simulink model "s_c_nbe_m32k"  (R2018a)
settings: Solver=VariableStepDiscrete  StartTime=0.0  StopTime=1000  RelTol=1e-3
undefined symbols (not defined in the file): fft_stages, n_taps, output_bits, pfb_coeff_gen_calc, xengbits
libraries: xbsIndex_r4 x23714, casper_library_misc x17, xps_library x4, casper_library_scopes x4, xbsReplacements_r4 x4
(part 152 of 171)

== system s_c_nbe_m32k/nb_pfb/pfb_fir_generic1/pfb_fir_taps/tap_delays/debus_web0 ==
  bus_in : Inport
  slice1 : xbsIndex_r4/Slice  nbits=1  boolean_output=on  mode=Upper Bit Location + Width  bit1=-107  base1=MSB of Input  bit0=0  base0=LSB of Input  dbl_ovrd=off  block_type=slice
  slice10 : xbsIndex_r4/Slice  nbits=1  boolean_output=on  mode=Upper Bit Location + Width  bit1=-98  base1=MSB of Input  bit0=0  base0=LSB of Input  dbl_ovrd=off  block_type=slice
  slice100 : xbsIndex_r4/Slice  nbits=1  boolean_output=on  mode=Upper Bit Location + Width  bit1=-8  base1=MSB of Input  bit0=0  base0=LSB of Input  dbl_ovrd=off  block_type=slice
  slice101 : xbsIndex_r4/Slice  nbits=1  boolean_output=on  mode=Upper Bit Location + Width  bit1=-7  base1=MSB of Input  bit0=0  base0=LSB of Input  dbl_ovrd=off  block_type=slice
  slice102 : xbsIndex_r4/Slice  nbits=1  boolean_output=on  mode=Upper Bit Location + Width  bit1=-6  base1=MSB of Input  bit0=0  base0=LSB of Input  dbl_ovrd=off  block_type=slice
  slice103 : xbsIndex_r4/Slice  nbits=1  boolean_output=on  mode=Upper Bit Location + Width  bit1=-5  base1=MSB of Input  bit0=0  base0=LSB of Input  dbl_ovrd=off  block_type=slice
  slice104 : xbsIndex_r4/Slice  nbits=1  boolean_output=on  mode=Upper Bit Location + Width  bit1=-4  base1=MSB of Input  bit0=0  base0=LSB of Input  dbl_ovrd=off  block_type=slice
  slice105 : xbsIndex_r4/Slice  nbits=1  boolean_output=on  mode=Upper Bit Location + Width  bit1=-3  base1=MSB of Input  bit0=0  base0=LSB of Input  dbl_ovrd=off  block_type=slice
  slice106 : xbsIndex_r4/Slice  nbits=1  boolean_output=on  mode=Upper Bit Location + Width  bit1=-2  base1=MSB of Input  bit0=0  base0=LSB of Input  dbl_ovrd=off  block_type=slice
  slice107 : xbsIndex_r4/Slice  nbits=1  boolean_output=on  mode=Upper Bit Location + Width  bit1=-1  base1=MSB of Input  bit0=0  base0=LSB of Input  dbl_ovrd=off  block_type=slice
  slice108 : xbsIndex_r4/Slice  nbits=1  boolean_output=on  mode=Upper Bit Location + Width  bit1=0  base1=MSB of Input  bit0=0  base0=LSB of Input  dbl_ovrd=off  block_type=slice
  slice11 : xbsIndex_r4/Slice  nbits=1  boolean_output=on  mode=Upper Bit Location + Width  bit1=-97  base1=MSB of Input  bit0=0  base0=LSB of Input  dbl_ovrd=off  block_type=slice
  slice12 : xbsIndex_r4/Slice  nbits=1  boolean_output=on  mode=Upper Bit Location + Width  bit1=-96  base1=MSB of Input  bit0=0  base0=LSB of Input  dbl_ovrd=off  block_type=slice
  slice13 : xbsIndex_r4/Slice  nbits=1  boolean_output=on  mode=Upper Bit Location + Width  bit1=-95  base1=MSB of Input  bit0=0  base0=LSB of Input  dbl_ovrd=off  block_type=slice
  slice14 : xbsIndex_r4/Slice  nbits=1  boolean_output=on  mode=Upper Bit Location + Width  bit1=-94  base1=MSB of Input  bit0=0  base0=LSB of Input  dbl_ovrd=off  block_type=slice
  slice15 : xbsIndex_r4/Slice  nbits=1  boolean_output=on  mode=Upper Bit Location + Width  bit1=-93  base1=MSB of Input  bit0=0  base0=LSB of Input  dbl_ovrd=off  block_type=slice
  slice16 : xbsIndex_r4/Slice  nbits=1  boolean_output=on  mode=Upper Bit Location + Width  bit1=-92  base1=MSB of Input  bit0=0  base0=LSB of Input  dbl_ovrd=off  block_type=slice
  slice17 : xbsIndex_r4/Slice  nbits=1  boolean_output=on  mode=Upper Bit Location + Width  bit1=-91  base1=MSB of Input  bit0=0  base0=LSB of Input  dbl_ovrd=off  block_type=slice
  slice18 : xbsIndex_r4/Slice  nbits=1  boolean_output=on  mode=Upper Bit Location + Width  bit1=-90  base1=MSB of Input  bit0=0  base0=LSB of Input  dbl_ovrd=off  block_type=slice
  slice19 : xbsIndex_r4/Slice  nbits=1  boolean_output=on  mode=Upper Bit Location + Width  bit1=-89  base1=MSB of Input  bit0=0  base0=LSB of Input  dbl_ovrd=off  block_type=slice
  slice2 : xbsIndex_r4/Slice  nbits=1  boolean_output=on  mode=Upper Bit Location + Width  bit1=-106  base1=MSB of Input  bit0=0  base0=LSB of Input  dbl_ovrd=off  block_type=slice
  slice20 : xbsIndex_r4/Slice  nbits=1  boolean_output=on  mode=Upper Bit Location + Width  bit1=-88  base1=MSB of Input  bit0=0  base0=LSB of Input  dbl_ovrd=off  block_type=slice
  slice21 : xbsIndex_r4/Slice  nbits=1  boolean_output=on  mode=Upper Bit Location + Width  bit1=-87  base1=MSB of Input  bit0=0  base0=LSB of Input  dbl_ovrd=off  block_type=slice
  slice22 : xbsIndex_r4/Slice  nbits=1  boolean_output=on  mode=Upper Bit Location + Width  bit1=-86  base1=MSB of Input  bit0=0  base0=LSB of Input  dbl_ovrd=off  block_type=slice
  slice23 : xbsIndex_r4/Slice  nbits=1  boolean_output=on  mode=Upper Bit Location + Width  bit1=-85  base1=MSB of Input  bit0=0  base0=LSB of Input  dbl_ovrd=off  block_type=slice
  slice24 : xbsIndex_r4/Slice  nbits=1  boolean_output=on  mode=Upper Bit Location + Width  bit1=-84  base1=MSB of Input  bit0=0  base0=LSB of Input  dbl_ovrd=off  block_type=slice
  slice25 : xbsIndex_r4/Slice  nbits=1  boolean_output=on  mode=Upper Bit Location + Width  bit1=-83  base1=MSB of Input  bit0=0  base0=LSB of Input  dbl_ovrd=off  block_type=slice
  slice26 : xbsIndex_r4/Slice  nbits=1  boolean_output=on  mode=Upper Bit Location + Width  bit1=-82  base1=MSB of Input  bit0=0  base0=LSB of Input  dbl_ovrd=off  block_type=slice
  slice27 : xbsIndex_r4/Slice  nbits=1  boolean_output=on  mode=Upper Bit Location + Width  bit1=-81  base1=MSB of Input  bit0=0  base0=LSB of Input  dbl_ovrd=off  block_type=slice
  slice28 : xbsIndex_r4/Slice  nbits=1  boolean_output=on  mode=Upper Bit Location + Width  bit1=-80  base1=MSB of Input  bit0=0  base0=LSB of Input  dbl_ovrd=off  block_type=slice
  slice29 : xbsIndex_r4/Slice  nbits=1  boolean_output=on  mode=Upper Bit Location + Width  bit1=-79  base1=MSB of Input  bit0=0  base0=LSB of Input  dbl_ovrd=off  block_type=slice
  slice3 : xbsIndex_r4/Slice  nbits=1  boolean_output=on  mode=Upper Bit Location + Width  bit1=-105  base1=MSB of Input  bit0=0  base0=LSB of Input  dbl_ovrd=off  block_type=slice
  slice30 : xbsIndex_r4/Slice  nbits=1  boolean_output=on  mode=Upper Bit Location + Width  bit1=-78  base1=MSB of Input  bit0=0  base0=LSB of Input  dbl_ovrd=off  block_type=slice
  slice31 : xbsIndex_r4/Slice  nbits=1  boolean_output=on  mode=Upper Bit Location + Width  bit1=-77  base1=MSB of Input  bit0=0  base0=LSB of Input  dbl_ovrd=off  block_type=slice
  slice32 : xbsIndex_r4/Slice  nbits=1  boolean_output=on  mode=Upper Bit Location + Width  bit1=-76  base1=MSB of Input  bit0=0  base0=LSB of Input  dbl_ovrd=off  block_type=slice
  slice33 : xbsIndex_r4/Slice  nbits=1  boolean_output=on  mode=Upper Bit Location + Width  bit1=-75  base1=MSB of Input  bit0=0  base0=LSB of Input  dbl_ovrd=off  block_type=slice
  slice34 : xbsIndex_r4/Slice  nbits=1  boolean_output=on  mode=Upper Bit Location + Width  bit1=-74  base1=MSB of Input  bit0=0  base0=LSB of Input  dbl_ovrd=off  block_type=slice
  slice35 : xbsIndex_r4/Slice  nbits=1  boolean_output=on  mode=Upper Bit Location + Width  bit1=-73  base1=MSB of Input  bit0=0  base0=LSB of Input  dbl_ovrd=off  block_type=slice
  slice36 : xbsIndex_r4/Slice  nbits=1  boolean_output=on  mode=Upper Bit Location + Width  bit1=-72  base1=MSB of Input  bit0=0  base0=LSB of Input  dbl_ovrd=off  block_type=slice
  slice37 : xbsIndex_r4/Slice  nbits=1  boolean_output=on  mode=Upper Bit Location + Width  bit1=-71  base1=MSB of Input  bit0=0  base0=LSB of Input  dbl_ovrd=off  block_type=slice
  slice38 : xbsIndex_r4/Slice  nbits=1  boolean_output=on  mode=Upper Bit Location + Width  bit1=-70  base1=MSB of Input  bit0=0  base0=LSB of Input  dbl_ovrd=off  block_type=slice
  slice39 : xbsIndex_r4/Slice  nbits=1  boolean_output=on  mode=Upper Bit Location + Width  bit1=-69  base1=MSB of Input  bit0=0  base0=LSB of Input  dbl_ovrd=off  block_type=slice
  slice4 : xbsIndex_r4/Slice  nbits=1  boolean_output=on  mode=Upper Bit Location + Width  bit1=-104  base1=MSB of Input  bit0=0  base0=LSB of Input  dbl_ovrd=off  block_type=slice
  slice40 : xbsIndex_r4/Slice  nbits=1  boolean_output=on  mode=Upper Bit Location + Width  bit1=-68  base1=MSB of Input  bit0=0  base0=LSB of Input  dbl_ovrd=off  block_type=slice
  slice41 : xbsIndex_r4/Slice  nbits=1  boolean_output=on  mode=Upper Bit Location + Width  bit1=-67  base1=MSB of Input  bit0=0  base0=LSB of Input  dbl_ovrd=off  block_type=slice
  slice42 : xbsIndex_r4/Slice  nbits=1  boolean_output=on  mode=Upper Bit Location + Width  bit1=-66  base1=MSB of Input  bit0=0  base0=LSB of Input  dbl_ovrd=off  block_type=slice
  slice43 : xbsIndex_r4/Slice  nbits=1  boolean_output=on  mode=Upper Bit Location + Width  bit1=-65  base1=MSB of Input  bit0=0  base0=LSB of Input  dbl_ovrd=off  block_type=slice
  slice44 : xbsIndex_r4/Slice  nbits=1  boolean_output=on  mode=Upper Bit Location + Width  bit1=-64  base1=MSB of Input  bit0=0  base0=LSB of Input  dbl_ovrd=off  block_type=slice
  slice45 : xbsIndex_r4/Slice  nbits=1  boolean_output=on  mode=Upper Bit Location + Width  bit1=-63  base1=MSB of Input  bit0=0  base0=LSB of Input  dbl_ovrd=off  block_type=slice
  slice46 : xbsIndex_r4/Slice  nbits=1  boolean_output=on  mode=Upper Bit Location + Width  bit1=-62  base1=MSB of Input  bit0=0  base0=LSB of Input  dbl_ovrd=off  block_type=slice
  slice47 : xbsIndex_r4/Slice  nbits=1  boolean_output=on  mode=Upper Bit Location + Width  bit1=-61  base1=MSB of Input  bit0=0  base0=LSB of Input  dbl_ovrd=off  block_type=slice
  slice48 : xbsIndex_r4/Slice  nbits=1  boolean_output=on  mode=Upper Bit Location + Width  bit1=-60  base1=MSB of Input  bit0=0  base0=LSB of Input  dbl_ovrd=off  block_type=slice
  slice49 : xbsIndex_r4/Slice  nbits=1  boolean_output=on  mode=Upper Bit Location + Width  bit1=-59  base1=MSB of Input  bit0=0  base0=LSB of Input  dbl_ovrd=off  block_type=slice
  slice5 : xbsIndex_r4/Slice  nbits=1  boolean_output=on  mode=Upper Bit Location + Width  bit1=-103  base1=MSB of Input  bit0=0  base0=LSB of Input  dbl_ovrd=off  block_type=slice
  slice50 : xbsIndex_r4/Slice  nbits=1  boolean_output=on  mode=Upper Bit Location + Width  bit1=-58  base1=MSB of Input  bit0=0  base0=LSB of Input  dbl_ovrd=off  block_type=slice
  slice51 : xbsIndex_r4/Slice  nbits=1  boolean_output=on  mode=Upper Bit Location + Width  bit1=-57  base1=MSB of Input  bit0=0  base0=LSB of Input  dbl_ovrd=off  block_type=slice
  slice52 : xbsIndex_r4/Slice  nbits=1  boolean_output=on  mode=Upper Bit Location + Width  bit1=-56  base1=MSB of Input  bit0=0  base0=LSB of Input  dbl_ovrd=off  block_type=slice
  slice53 : xbsIndex_r4/Slice  nbits=1  boolean_output=on  mode=Upper Bit Location + Width  bit1=-55  base1=MSB of Input  bit0=0  base0=LSB of Input  dbl_ovrd=off  block_type=slice
  slice54 : xbsIndex_r4/Slice  nbits=1  boolean_output=on  mode=Upper Bit Location + Width  bit1=-54  base1=MSB of Input  bit0=0  base0=LSB of Input  dbl_ovrd=off  block_type=slice
  slice55 : xbsIndex_r4/Slice  nbits=1  boolean_output=on  mode=Upper Bit Location + Width  bit1=-53  base1=MSB of Input  bit0=0  base0=LSB of Input  dbl_ovrd=off  block_type=slice
  slice56 : xbsIndex_r4/Slice  nbits=1  boolean_output=on  mode=Upper Bit Location + Width  bit1=-52  base1=MSB of Input  bit0=0  base0=LSB of Input  dbl_ovrd=off  block_type=slice
  slice57 : xbsIndex_r4/Slice  nbits=1  boolean_output=on  mode=Upper Bit Location + Width  bit1=-51  base1=MSB of Input  bit0=0  base0=LSB of Input  dbl_ovrd=off  block_type=slice
  slice58 : xbsIndex_r4/Slice  nbits=1  boolean_output=on  mode=Upper Bit Location + Width  bit1=-50  base1=MSB of Input  bit0=0  base0=LSB of Input  dbl_ovrd=off  block_type=slice
  slice59 : xbsIndex_r4/Slice  nbits=1  boolean_output=on  mode=Upper Bit Location + Width  bit1=-49  base1=MSB of Input  bit0=0  base0=LSB of Input  dbl_ovrd=off  block_type=slice
  slice6 : xbsIndex_r4/Slice  nbits=1  boolean_output=on  mode=Upper Bit Location + Width  bit1=-102  base1=MSB of Input  bit0=0  base0=LSB of Input  dbl_ovrd=off  block_type=slice
  slice60 : xbsIndex_r4/Slice  nbits=1  boolean_output=on  mode=Upper Bit Location + Width  bit1=-48  base1=MSB of Input  bit0=0  base0=LSB of Input  dbl_ovrd=off  block_type=slice
  slice61 : xbsIndex_r4/Slice  nbits=1  boolean_output=on  mode=Upper Bit Location + Width  bit1=-47  base1=MSB of Input  bit0=0  base0=LSB of Input  dbl_ovrd=off  block_type=slice
  slice62 : xbsIndex_r4/Slice  nbits=1  boolean_output=on  mode=Upper Bit Location + Width  bit1=-46  base1=MSB of Input  bit0=0  base0=LSB of Input  dbl_ovrd=off  block_type=slice
  slice63 : xbsIndex_r4/Slice  nbits=1  boolean_output=on  mode=Upper Bit Location + Width  bit1=-45  base1=MSB of Input  bit0=0  base0=LSB of Input  dbl_ovrd=off  block_type=slice
  slice64 : xbsIndex_r4/Slice  nbits=1  boolean_output=on  mode=Upper Bit Location + Width  bit1=-44  base1=MSB of Input  bit0=0  base0=LSB of Input  dbl_ovrd=off  block_type=slice
  slice65 : xbsIndex_r4/Slice  nbits=1  boolean_output=on  mode=Upper Bit Location + Width  bit1=-43  base1=MSB of Input  bit0=0  base0=LSB of Input  dbl_ovrd=off  block_type=slice
  slice66 : xbsIndex_r4/Slice  nbits=1  boolean_output=on  mode=Upper Bit Location + Width  bit1=-42  base1=MSB of Input  bit0=0  base0=LSB of Input  dbl_ovrd=off  block_type=slice
  slice67 : xbsIndex_r4/Slice  nbits=1  boolean_output=on  mode=Upper Bit Location + Width  bit1=-41  base1=MSB of Input  bit0=0  base0=LSB of Input  dbl_ovrd=off  block_type=slice
  slice68 : xbsIndex_r4/Slice  nbits=1  boolean_output=on  mode=Upper Bit Location + Width  bit1=-40  base1=MSB of Input  bit0=0  base0=LSB of Input  dbl_ovrd=off  block_type=slice
  slice69 : xbsIndex_r4/Slice  nbits=1  boolean_output=on  mode=Upper Bit Location + Width  bit1=-39  base1=MSB of Input  bit0=0  base0=LSB of Input  dbl_ovrd=off  block_type=slice
  slice7 : xbsIndex_r4/Slice  nbits=1  boolean_output=on  mode=Upper Bit Location + Width  bit1=-101  base1=MSB of Input  bit0=0  base0=LSB of Input  dbl_ovrd=off  block_type=slice
  slice70 : xbsIndex_r4/Slice  nbits=1  boolean_output=on  mode=Upper Bit Location + Width  bit1=-38  base1=MSB of Input  bit0=0  base0=LSB of Input  dbl_ovrd=off  block_type=slice
  slice71 : xbsIndex_r4/Slice  nbits=1  boolean_output=on  mode=Upper Bit Location + Width  bit1=-37  base1=MSB of Input  bit0=0  base0=LSB of Input  dbl_ovrd=off  block_type=slice
  slice72 : xbsIndex_r4/Slice  nbits=1  boolean_output=on  mode=Upper Bit Location + Width  bit1=-36  base1=MSB of Input  bit0=0  base0=LSB of Input  dbl_ovrd=off  block_type=slice
  slice73 : xbsIndex_r4/Slice  nbits=1  boolean_output=on  mode=Upper Bit Location + Width  bit1=-35  base1=MSB of Input  bit0=0  base0=LSB of Input  dbl_ovrd=off  block_type=slice
  slice74 : xbsIndex_r4/Slice  nbits=1  boolean_output=on  mode=Upper Bit Location + Width  bit1=-34  base1=MSB of Input  bit0=0  base0=LSB of Input  dbl_ovrd=off  block_type=slice
  slice75 : xbsIndex_r4/Slice  nbits=1  boolean_output=on  mode=Upper Bit Location + Width  bit1=-33  base1=MSB of Input  bit0=0  base0=LSB of Input  dbl_ovrd=off  block_type=slice
  slice76 : xbsIndex_r4/Slice  nbits=1  boolean_output=on  mode=Upper Bit Location + Width  bit1=-32  base1=MSB of Input  bit0=0  base0=LSB of Input  dbl_ovrd=off  block_type=slice
  slice77 : xbsIndex_r4/Slice  nbits=1  boolean_output=on  mode=Upper Bit Location + Width  bit1=-31  base1=MSB of Input  bit0=0  base0=LSB of Input  dbl_ovrd=off  block_type=slice
  slice78 : xbsIndex_r4/Slice  nbits=1  boolean_output=on  mode=Upper Bit Location + Width  bit1=-30  base1=MSB of Input  bit0=0  base0=LSB of Input  dbl_ovrd=off  block_type=slice
  slice79 : xbsIndex_r4/Slice  nbits=1  boolean_output=on  mode=Upper Bit Location + Width  bit1=-29  base1=MSB of Input  bit0=0  base0=LSB of Input  dbl_ovrd=off  block_type=slice
  slice8 : xbsIndex_r4/Slice  nbits=1  boolean_output=on  mode=Upper Bit Location + Width  bit1=-100  base1=MSB of Input  bit0=0  base0=LSB of Input  dbl_ovrd=off  block_type=slice
  slice80 : xbsIndex_r4/Slice  nbits=1  boolean_output=on  mode=Upper Bit Location + Width  bit1=-28  base1=MSB of Input  bit0=0  base0=LSB of Input  dbl_ovrd=off  block_type=slice
  slice81 : xbsIndex_r4/Slice  nbits=1  boolean_output=on  mode=Upper Bit Location + Width  bit1=-27  base1=MSB of Input  bit0=0  base0=LSB of Input  dbl_ovrd=off  block_type=slice
  slice82 : xbsIndex_r4/Slice  nbits=1  boolean_output=on  mode=Upper Bit Location + Width  bit1=-26  base1=MSB of Input  bit0=0  base0=LSB of Input  dbl_ovrd=off  block_type=slice
  slice83 : xbsIndex_r4/Slice  nbits=1  boolean_output=on  mode=Upper Bit Location + Width  bit1=-25  base1=MSB of Input  bit0=0  base0=LSB of Input  dbl_ovrd=off  block_type=slice
  slice84 : xbsIndex_r4/Slice  nbits=1  boolean_output=on  mode=Upper Bit Location + Width  bit1=-24  base1=MSB of Input  bit0=0  base0=LSB of Input  dbl_ovrd=off  block_type=slice
  slice85 : xbsIndex_r4/Slice  nbits=1  boolean_output=on  mode=Upper Bit Location + Width  bit1=-23  base1=MSB of Input  bit0=0  base0=LSB of Input  dbl_ovrd=off  block_type=slice
  slice86 : xbsIndex_r4/Slice  nbits=1  boolean_output=on  mode=Upper Bit Location + Width  bit1=-22  base1=MSB of Input  bit0=0  base0=LSB of Input  dbl_ovrd=off  block_type=slice
  slice87 : xbsIndex_r4/Slice  nbits=1  boolean_output=on  mode=Upper Bit Location + Width  bit1=-21  base1=MSB of Input  bit0=0  base0=LSB of Input  dbl_ovrd=off  block_type=slice
  slice88 : xbsIndex_r4/Slice  nbits=1  boolean_output=on  mode=Upper Bit Location + Width  bit1=-20  base1=MSB of Input  bit0=0  base0=LSB of Input  dbl_ovrd=off  block_type=slice
  slice89 : xbsIndex_r4/Slice  nbits=1  boolean_output=on  mode=Upper Bit Location + Width  bit1=-19  base1=MSB of Input  bit0=0  base0=LSB of Input  dbl_ovrd=off  block_type=slice
  slice9 : xbsIndex_r4/Slice  nbits=1  boolean_output=on  mode=Upper Bit Location + Width  bit1=-99  base1=MSB of Input  bit0=0  base0=LSB of Input  dbl_ovrd=off  block_type=slice
  slice90 : xbsIndex_r4/Slice  nbits=1  boolean_output=on  mode=Upper Bit Location + Width  bit1=-18  base1=MSB of Input  bit0=0  base0=LSB of Input  dbl_ovrd=off  block_type=slice
  slice91 : xbsIndex_r4/Slice  nbits=1  boolean_output=on  mode=Upper Bit Location + Width  bit1=-17  base1=MSB of Input  bit0=0  base0=LSB of Input  dbl_ovrd=off  block_type=slice
  slice92 : xbsIndex_r4/Slice  nbits=1  boolean_output=on  mode=Upper Bit Location + Width  bit1=-16  base1=MSB of Input  bit0=0  base0=LSB of Input  dbl_ovrd=off  block_type=slice
  slice93 : xbsIndex_r4/Slice  nbits=1  boolean_output=on  mode=Upper Bit Location + Width  bit1=-15  base1=MSB of Input  bit0=0  base0=LSB of Input  dbl_ovrd=off  block_type=slice
  slice94 : xbsIndex_r4/Slice  nbits=1  boolean_output=on  mode=Upper Bit Location + Width  bit1=-14  base1=MSB of Input  bit0=0  base0=LSB of Input  dbl_ovrd=off  block_type=slice
  slice95 : xbsIndex_r4/Slice  nbits=1  boolean_output=on  mode=Upper Bit Location + Width  bit1=-13  base1=MSB of Input  bit0=0  base0=LSB of Input  dbl_ovrd=off  block_type=slice
  slice96 : xbsIndex_r4/Slice  nbits=1  boolean_output=on  mode=Upper Bit Location + Width  bit1=-12  base1=MSB of Input  bit0=0  base0=LSB of Input  dbl_ovrd=off  block_type=slice
  slice97 : xbsIndex_r4/Slice  nbits=1  boolean_output=on  mode=Upper Bit Location + Width  bit1=-11  base1=MSB of Input  bit0=0  base0=LSB of Input  dbl_ovrd=off  block_type=slice
  slice98 : xbsIndex_r4/Slice  nbits=1  boolean_output=on  mode=Upper Bit Location + Width  bit1=-10  base1=MSB of Input  bit0=0  base0=LSB of Input  dbl_ovrd=off  block_type=slice
  slice99 : xbsIndex_r4/Slice  nbits=1  boolean_output=on  mode=Upper Bit Location + Width  bit1=-9  base1=MSB of Input  bit0=0  base0=LSB of Input  dbl_ovrd=off  block_type=slice
  msb_out108 : Outport
  out107 : Outport  Port=2
  out106 : Outport  Port=3
  out105 : Outport  Port=4
  out104 : Outport  Port=5
  out103 : Outport  Port=6
  out102 : Outport  Port=7
  out101 : Outport  Port=8
  out100 : Outport  Port=9
  out99 : Outport  Port=10
  out98 : Outport  Port=11
  out97 : Outport  Port=12
  out96 : Outport  Port=13
  out95 : Outport  Port=14
  out94 : Outport  Port=15
  out93 : Outport  Port=16
  out92 : Outport  Port=17
  out91 : Outport  Port=18
  out90 : Outport  Port=19
  out89 : Outport  Port=20
  out88 : Outport  Port=21
  out87 : Outport  Port=22
  out86 : Outport  Port=23
  out85 : Outport  Port=24
  out84 : Outport  Port=25
  out83 : Outport  Port=26
  out82 : Outport  Port=27
  out81 : Outport  Port=28
  out80 : Outport  Port=29
  out79 : Outport  Port=30
  out78 : Outport  Port=31
  out77 : Outport  Port=32
  out76 : Outport  Port=33
  out75 : Outport  Port=34
  out74 : Outport  Port=35
  out73 : Outport  Port=36
  out72 : Outport  Port=37
  out71 : Outport  Port=38
  out70 : Outport  Port=39
  out69 : Outport  Port=40
  out68 : Outport  Port=41
  out67 : Outport  Port=42
  out66 : Outport  Port=43
  out65 : Outport  Port=44
  out64 : Outport  Port=45
  out63 : Outport  Port=46
  out62 : Outport  Port=47
  out61 : Outport  Port=48
  out60 : Outport  Port=49
  out59 : Outport  Port=50
  out58 : Outport  Port=51
  out57 : Outport  Port=52
  out56 : Outport  Port=53
  out55 : Outport  Port=54
  out54 : Outport  Port=55
  out53 : Outport  Port=56
  out52 : Outport  Port=57
  out51 : Outport  Port=58
  out50 : Outport  Port=59
  out49 : Outport  Port=60
  out48 : Outport  Port=61
  out47 : Outport  Port=62
  out46 : Outport  Port=63
  out45 : Outport  Port=64
  out44 : Outport  Port=65
  out43 : Outport  Port=66
  out42 : Outport  Port=67
  out41 : Outport  Port=68
  out40 : Outport  Port=69
  out39 : Outport  Port=70
  out38 : Outport  Port=71
  out37 : Outport  Port=72
  out36 : Outport  Port=73
  out35 : Outport  Port=74
  out34 : Outport  Port=75
  out33 : Outport  Port=76
  out32 : Outport  Port=77
  out31 : Outport  Port=78
  out30 : Outport  Port=79
  out29 : Outport  Port=80
  out28 : Outport  Port=81
  out27 : Outport  Port=82
  out26 : Outport  Port=83
  out25 : Outport  Port=84
  out24 : Outport  Port=85
  out23 : Outport  Port=86
  out22 : Outport  Port=87
  out21 : Outport  Port=88
  out20 : Outport  Port=89
  out19 : Outport  Port=90
  out18 : Outport  Port=91
  out17 : Outport  Port=92
  out16 : Outport  Port=93
  out15 : Outport  Port=94
  out14 : Outport  Port=95
  out13 : Outport  Port=96
  out12 : Outport  Port=97
  out11 : Outport  Port=98
  out10 : Outport  Port=99
  out9 : Outport  Port=100
  out8 : Outport  Port=101
  out7 : Outport  Port=102
  out6 : Outport  Port=103
  out5 : Outport  Port=104
  out4 : Outport  Port=105
  out3 : Outport  Port=106
  out2 : Outport  Port=107
  lsb_out1 : Outport  Port=108
  wires:
  bus_in/1 -> slice108/1, slice107/1, slice106/1, slice105/1, slice104/1, slice103/1, slice102/1, slice101/1, slice100/1, slice99/1, slice98/1, slice97/1, slice96/1, slice95/1, slice94/1, slice93/1, slice92/1, slice91/1, slice90/1, slice89/1, slice88/1, slice87/1, slice86/1, slice85/1, slice84/1, slice83/1, slice82/1, slice81/1, slice80/1, slice79/1, slice78/1, slice77/1, slice76/1, slice75/1, slice74/1, slice73/1, slice72/1, slice71/1, slice70/1, slice69/1, slice68/1, slice67/1, slice66/1, slice65/1, slice64/1, slice63/1, slice62/1, slice61/1, slice60/1, slice59/1, slice58/1, slice57/1, slice56/1, slice55/1, slice54/1, slice53/1, slice52/1, slice51/1, slice50/1, slice49/1, slice48/1, slice47/1, slice46/1, slice45/1, slice44/1, slice43/1, slice42/1, slice41/1, slice40/1, slice39/1, slice38/1, slice37/1, slice36/1, slice35/1, slice34/1, slice33/1, slice32/1, slice31/1, slice30/1, slice29/1, slice28/1, slice27/1, slice26/1, slice25/1, slice24/1, slice23/1, slice22/1, slice21/1, slice20/1, slice19/1, slice18/1, slice17/1, slice16/1, slice15/1, slice14/1, slice13/1, slice12/1, slice11/1, slice10/1, slice9/1, slice8/1, slice7/1, slice6/1, slice5/1, slice4/1, slice3/1, slice2/1, slice1/1
  slice108/1 -> msb_out108/1
  slice107/1 -> out107/1
  slice106/1 -> out106/1
  slice105/1 -> out105/1
  slice104/1 -> out104/1
  slice103/1 -> out103/1
  slice102/1 -> out102/1
  slice101/1 -> out101/1
  slice100/1 -> out100/1
  slice99/1 -> out99/1
  slice98/1 -> out98/1
  slice97/1 -> out97/1
  slice96/1 -> out96/1
  slice95/1 -> out95/1
  slice94/1 -> out94/1
  slice93/1 -> out93/1
  slice92/1 -> out92/1
  slice91/1 -> out91/1
  slice90/1 -> out90/1
  slice89/1 -> out89/1
  slice88/1 -> out88/1
  slice87/1 -> out87/1
  slice86/1 -> out86/1
  slice85/1 -> out85/1
  slice84/1 -> out84/1
  slice83/1 -> out83/1
  slice82/1 -> out82/1
  slice81/1 -> out81/1
  slice80/1 -> out80/1
  slice79/1 -> out79/1
  slice78/1 -> out78/1
  slice77/1 -> out77/1
  slice76/1 -> out76/1
  slice75/1 -> out75/1
  slice74/1 -> out74/1
  slice73/1 -> out73/1
  slice72/1 -> out72/1
  slice71/1 -> out71/1
  slice70/1 -> out70/1
  slice69/1 -> out69/1
  slice68/1 -> out68/1
  slice67/1 -> out67/1
  slice66/1 -> out66/1
  slice65/1 -> out65/1
  slice64/1 -> out64/1
  slice63/1 -> out63/1
  slice62/1 -> out62/1
  slice61/1 -> out61/1
  slice60/1 -> out60/1
  slice59/1 -> out59/1
  slice58/1 -> out58/1
  slice57/1 -> out57/1
  slice56/1 -> out56/1
  slice55/1 -> out55/1
  slice54/1 -> out54/1
  slice53/1 -> out53/1
  slice52/1 -> out52/1
  slice51/1 -> out51/1
  slice50/1 -> out50/1
  slice49/1 -> out49/1
  slice48/1 -> out48/1
  slice47/1 -> out47/1
  slice46/1 -> out46/1
  slice45/1 -> out45/1
  slice44/1 -> out44/1
  slice43/1 -> out43/1
  slice42/1 -> out42/1
  slice41/1 -> out41/1
  slice40/1 -> out40/1
  slice39/1 -> out39/1
  slice38/1 -> out38/1
  slice37/1 -> out37/1
  slice36/1 -> out36/1
  slice35/1 -> out35/1
  slice34/1 -> out34/1
  slice33/1 -> out33/1
  slice32/1 -> out32/1
  slice31/1 -> out31/1
  slice30/1 -> out30/1
  slice29/1 -> out29/1
  slice28/1 -> out28/1
  slice27/1 -> out27/1
  slice26/1 -> out26/1
  slice25/1 -> out25/1
  slice24/1 -> out24/1
  slice23/1 -> out23/1
  slice22/1 -> out22/1
  slice21/1 -> out21/1
  slice20/1 -> out20/1
  slice19/1 -> out19/1
  slice18/1 -> out18/1
  slice17/1 -> out17/1
  slice16/1 -> out16/1
  slice15/1 -> out15/1
  slice14/1 -> out14/1
  slice13/1 -> out13/1
  slice12/1 -> out12/1
  slice11/1 -> out11/1
  slice10/1 -> out10/1
  slice9/1 -> out9/1
  slice8/1 -> out8/1
  slice7/1 -> out7/1
  slice6/1 -> out6/1
  slice5/1 -> out5/1
  slice4/1 -> out4/1
  slice3/1 -> out3/1
  slice2/1 -> out2/1
  slice1/1 -> lsb_out1/1

== system s_c_nbe_m32k/nb_pfb/pfb_fir_generic1/pfb_fir_taps/tap_delays/rep_addra0 ==
  in : Inport
  bussify : Subsystem  mask(bus_create){inputNum=108}
      mask prompts: inputNum "Number of inputs:"
      mask init:
      | bus_create_init(gcb,...
      |     'inputNum', inputNum);
  din0_0 : xbsIndex_r4/Delay  rst=off  infoeditControl=Selection of Reset will increase slice count due to use of real FFs and instead of SRLs  en=off  latency=1  reg_retiming=off  dbl_ovrd=off  block_type=delay
  din0_1 : xbsIndex_r4/Delay  rst=off  infoeditControl=Selection of Reset will increase slice count due to use of real FFs and instead of SRLs  en=off  latency=1  reg_retiming=off  dbl_ovrd=off  block_type=delay
  din0_2 : xbsIndex_r4/Delay  rst=off  infoeditControl=Selection of Reset will increase slice count due to use of real FFs and instead of SRLs  en=off  latency=1  reg_retiming=off  dbl_ovrd=off  block_type=delay
  din1_{0..11} (12 alike) : xbsIndex_r4/Delay  rst=off  infoeditControl=Selection of Reset will increase slice count due to use of real FFs and instead of SRLs  en=off  latency=1  reg_retiming=off  dbl_ovrd=off  block_type=delay
  din2_{0..47} (48 alike) : xbsIndex_r4/Delay  rst=off  infoeditControl=Selection of Reset will increase slice count due to use of real FFs and instead of SRLs  en=off  latency=1  reg_retiming=off  dbl_ovrd=off  block_type=delay
  din3_{0..107} (108 alike) : xbsIndex_r4/Delay  rst=off  infoeditControl=Selection of Reset will increase slice count due to use of real FFs and instead of SRLs  en=off  latency=1  reg_retiming=off  dbl_ovrd=off  block_type=delay
  out : Outport
  wires:
  in/1 -> din0_0/1, din0_1/1, din0_2/1
  din0_0/1 -> din1_0/1, din1_3/1, din1_6/1, din1_9/1
  din0_1/1 -> din1_1/1, din1_4/1, din1_7/1, din1_10/1
  din0_2/1 -> din1_2/1, din1_5/1, din1_8/1, din1_11/1
  din1_0/1 -> din2_0/1, din2_12/1, din2_24/1, din2_36/1
  din1_1/1 -> din2_1/1, din2_13/1, din2_25/1, din2_37/1
  din1_2/1 -> din2_2/1, din2_14/1, din2_26/1, din2_38/1
  din1_3/1 -> din2_3/1, din2_15/1, din2_27/1, din2_39/1
  din1_4/1 -> din2_4/1, din2_16/1, din2_28/1, din2_40/1
  din1_5/1 -> din2_5/1, din2_17/1, din2_29/1, din2_41/1
  din1_6/1 -> din2_6/1, din2_18/1, din2_30/1, din2_42/1
  din1_7/1 -> din2_7/1, din2_19/1, din2_31/1, din2_43/1
  din1_8/1 -> din2_8/1, din2_20/1, din2_32/1, din2_44/1
  din1_9/1 -> din2_9/1, din2_21/1, din2_33/1, din2_45/1
  din1_10/1 -> din2_10/1, din2_22/1, din2_34/1, din2_46/1
  din1_11/1 -> din2_11/1, din2_23/1, din2_35/1, din2_47/1
  din2_0/1 -> din3_0/1, din3_48/1, din3_96/1
  din2_1/1 -> din3_1/1, din3_49/1, din3_97/1
  din2_2/1 -> din3_2/1, din3_50/1, din3_98/1
  din2_3/1 -> din3_3/1, din3_51/1, din3_99/1
  din2_4/1 -> din3_4/1, din3_52/1, din3_100/1
  din2_5/1 -> din3_5/1, din3_53/1, din3_101/1
  din2_6/1 -> din3_6/1, din3_54/1, din3_102/1
  din2_7/1 -> din3_7/1, din3_55/1, din3_103/1
  din2_8/1 -> din3_8/1, din3_56/1, din3_104/1
  din2_9/1 -> din3_9/1, din3_57/1, din3_105/1
  din2_10/1 -> din3_10/1, din3_58/1, din3_106/1
  din2_11/1 -> din3_11/1, din3_59/1, din3_107/1
  din2_12/1 -> din3_12/1, din3_60/1
  din2_13/1 -> din3_13/1, din3_61/1
  din2_14/1 -> din3_14/1, din3_62/1
  din2_15/1 -> din3_15/1, din3_63/1
  din2_16/1 -> din3_16/1, din3_64/1
  din2_17/1 -> din3_17/1, din3_65/1
  din2_18/1 -> din3_18/1, din3_66/1
  din2_19/1 -> din3_19/1, din3_67/1
  din2_20/1 -> din3_20/1, din3_68/1
  din2_21/1 -> din3_21/1, din3_69/1
  din2_22/1 -> din3_22/1, din3_70/1
  din2_23/1 -> din3_23/1, din3_71/1
  din2_24/1 -> din3_24/1, din3_72/1
  din2_25/1 -> din3_25/1, din3_73/1
  din2_26/1 -> din3_26/1, din3_74/1
  din2_27/1 -> din3_27/1, din3_75/1
  din2_28/1 -> din3_28/1, din3_76/1
  din2_29/1 -> din3_29/1, din3_77/1
  din2_30/1 -> din3_30/1, din3_78/1
  din2_31/1 -> din3_31/1, din3_79/1
  din2_32/1 -> din3_32/1, din3_80/1
  din2_33/1 -> din3_33/1, din3_81/1
  din2_34/1 -> din3_34/1, din3_82/1
  din2_35/1 -> din3_35/1, din3_83/1
  din2_36/1 -> din3_36/1, din3_84/1
  din2_37/1 -> din3_37/1, din3_85/1
  din2_38/1 -> din3_38/1, din3_86/1
  din2_39/1 -> din3_39/1, din3_87/1
  din2_40/1 -> din3_40/1, din3_88/1
  din2_41/1 -> din3_41/1, din3_89/1
  din2_42/1 -> din3_42/1, din3_90/1
  din2_43/1 -> din3_43/1, din3_91/1
  din2_44/1 -> din3_44/1, din3_92/1
  din2_45/1 -> din3_45/1, din3_93/1
  din2_46/1 -> din3_46/1, din3_94/1
  din2_47/1 -> din3_47/1, din3_95/1
  din3_0/1 -> bussify/1(in1)
  din3_1/1 -> bussify/2(in2)
  din3_2/1 -> bussify/3(in3)
  din3_3/1 -> bussify/4(in4)
  din3_4/1 -> bussify/5(in5)
  din3_5/1 -> bussify/6(in6)
  din3_6/1 -> bussify/7(in7)
  din3_7/1 -> bussify/8(in8)
  din3_8/1 -> bussify/9(in9)
  din3_9/1 -> bussify/10(in10)
  din3_10/1 -> bussify/11(in11)
  din3_11/1 -> bussify/12(in12)
  din3_12/1 -> bussify/13(in13)
  din3_13/1 -> bussify/14(in14)
  din3_14/1 -> bussify/15(in15)
  din3_15/1 -> bussify/16(in16)
  din3_16/1 -> bussify/17(in17)
  din3_17/1 -> bussify/18(in18)
  din3_18/1 -> bussify/19(in19)
  din3_19/1 -> bussify/20(in20)
  din3_20/1 -> bussify/21(in21)
  din3_21/1 -> bussify/22(in22)
  din3_22/1 -> bussify/23(in23)
  din3_23/1 -> bussify/24(in24)
  din3_24/1 -> bussify/25(in25)
  din3_25/1 -> bussify/26(in26)
  din3_26/1 -> bussify/27(in27)
  din3_27/1 -> bussify/28(in28)
  din3_28/1 -> bussify/29(in29)
  din3_29/1 -> bussify/30(in30)
  din3_30/1 -> bussify/31(in31)
  din3_31/1 -> bussify/32(in32)
  din3_32/1 -> bussify/33(in33)
  din3_33/1 -> bussify/34(in34)
  din3_34/1 -> bussify/35(in35)
  din3_35/1 -> bussify/36(in36)
  din3_36/1 -> bussify/37(in37)
  din3_37/1 -> bussify/38(in38)
  din3_38/1 -> bussify/39(in39)
  din3_39/1 -> bussify/40(in40)
  din3_40/1 -> bussify/41(in41)
  din3_41/1 -> bussify/42(in42)
  din3_42/1 -> bussify/43(in43)
  din3_43/1 -> bussify/44(in44)
  din3_44/1 -> bussify/45(in45)
  din3_45/1 -> bussify/46(in46)
  din3_46/1 -> bussify/47(in47)
  din3_47/1 -> bussify/48(in48)
  din3_48/1 -> bussify/49(in49)
  din3_49/1 -> bussify/50(in50)
  din3_50/1 -> bussify/51(in51)
  din3_51/1 -> bussify/52(in52)
  din3_52/1 -> bussify/53(in53)
  din3_53/1 -> bussify/54(in54)
  din3_54/1 -> bussify/55(in55)
  din3_55/1 -> bussify/56(in56)
  din3_56/1 -> bussify/57(in57)
  din3_57/1 -> bussify/58(in58)
  din3_58/1 -> bussify/59(in59)
  din3_59/1 -> bussify/60(in60)
  din3_60/1 -> bussify/61(in61)
  din3_61/1 -> bussify/62(in62)
  din3_62/1 -> bussify/63(in63)
  din3_63/1 -> bussify/64(in64)
  din3_64/1 -> bussify/65(in65)
  din3_65/1 -> bussify/66(in66)
  din3_66/1 -> bussify/67(in67)
  din3_67/1 -> bussify/68(in68)
  din3_68/1 -> bussify/69(in69)
  din3_69/1 -> bussify/70(in70)
  din3_70/1 -> bussify/71(in71)
  din3_71/1 -> bussify/72(in72)
  din3_72/1 -> bussify/73(in73)
  din3_73/1 -> bussify/74(in74)
  din3_74/1 -> bussify/75(in75)
  din3_75/1 -> bussify/76(in76)
  din3_76/1 -> bussify/77(in77)
  din3_77/1 -> bussify/78(in78)
  din3_78/1 -> bussify/79(in79)
  din3_79/1 -> bussify/80(in80)
  din3_80/1 -> bussify/81(in81)
  din3_81/1 -> bussify/82(in82)
  din3_82/1 -> bussify/83(in83)
  din3_83/1 -> bussify/84(in84)
  din3_84/1 -> bussify/85(in85)
  din3_85/1 -> bussify/86(in86)
  din3_86/1 -> bussify/87(in87)
  din3_87/1 -> bussify/88(in88)
  din3_88/1 -> bussify/89(in89)
  din3_89/1 -> bussify/90(in90)
  din3_90/1 -> bussify/91(in91)
  din3_91/1 -> bussify/92(in92)
  din3_92/1 -> bussify/93(in93)
  din3_93/1 -> bussify/94(in94)
  din3_94/1 -> bussify/95(in95)
  din3_95/1 -> bussify/96(in96)
  din3_96/1 -> bussify/97(in97)
  din3_97/1 -> bussify/98(in98)
  din3_98/1 -> bussify/99(in99)
  din3_99/1 -> bussify/100(in100)
  din3_100/1 -> bussify/101(in101)
  din3_101/1 -> bussify/102(in102)
  din3_102/1 -> bussify/103(in103)
  din3_103/1 -> bussify/104(in104)
  din3_104/1 -> bussify/105(in105)
  din3_105/1 -> bussify/106(in106)
  din3_106/1 -> bussify/107(in107)
  din3_107/1 -> bussify/108(in108)
  bussify/1(bus_out) -> out/1

== system s_c_nbe_m32k/nb_pfb/pfb_fir_generic1/pfb_fir_taps/tap_delays/rep_addrb0 ==
  in : Inport
  bussify : Subsystem  mask(bus_create){inputNum=108}
      mask prompts: inputNum "Number of inputs:"
      mask init:
      | bus_create_init(gcb,...
      |     'inputNum', inputNum);
  din0_0 : xbsIndex_r4/Delay  rst=off  infoeditControl=Selection of Reset will increase slice count due to use of real FFs and instead of SRLs  en=off  latency=1  reg_retiming=off  dbl_ovrd=off  block_type=delay
  din0_1 : xbsIndex_r4/Delay  rst=off  infoeditControl=Selection of Reset will increase slice count due to use of real FFs and instead of SRLs  en=off  latency=1  reg_retiming=off  dbl_ovrd=off  block_type=delay
  din0_2 : xbsIndex_r4/Delay  rst=off  infoeditControl=Selection of Reset will increase slice count due to use of real FFs and instead of SRLs  en=off  latency=1  reg_retiming=off  dbl_ovrd=off  block_type=delay
  din1_{0..11} (12 alike) : xbsIndex_r4/Delay  rst=off  infoeditControl=Selection of Reset will increase slice count due to use of real FFs and instead of SRLs  en=off  latency=1  reg_retiming=off  dbl_ovrd=off  block_type=delay
  din2_{0..47} (48 alike) : xbsIndex_r4/Delay  rst=off  infoeditControl=Selection of Reset will increase slice count due to use of real FFs and instead of SRLs  en=off  latency=1  reg_retiming=off  dbl_ovrd=off  block_type=delay
  din3_{0..107} (108 alike) : xbsIndex_r4/Delay  rst=off  infoeditControl=Selection of Reset will increase slice count due to use of real FFs and instead of SRLs  en=off  latency=1  reg_retiming=off  dbl_ovrd=off  block_type=delay
  out : Outport
  wires:
  in/1 -> din0_0/1, din0_1/1, din0_2/1
  din0_0/1 -> din1_0/1, din1_3/1, din1_6/1, din1_9/1
  din0_1/1 -> din1_1/1, din1_4/1, din1_7/1, din1_10/1
  din0_2/1 -> din1_2/1, din1_5/1, din1_8/1, din1_11/1
  din1_0/1 -> din2_0/1, din2_12/1, din2_24/1, din2_36/1
  din1_1/1 -> din2_1/1, din2_13/1, din2_25/1, din2_37/1
  din1_2/1 -> din2_2/1, din2_14/1, din2_26/1, din2_38/1
  din1_3/1 -> din2_3/1, din2_15/1, din2_27/1, din2_39/1
  din1_4/1 -> din2_4/1, din2_16/1, din2_28/1, din2_40/1
  din1_5/1 -> din2_5/1, din2_17/1, din2_29/1, din2_41/1
  din1_6/1 -> din2_6/1, din2_18/1, din2_30/1, din2_42/1
  din1_7/1 -> din2_7/1, din2_19/1, din2_31/1, din2_43/1
  din1_8/1 -> din2_8/1, din2_20/1, din2_32/1, din2_44/1
  din1_9/1 -> din2_9/1, din2_21/1, din2_33/1, din2_45/1
  din1_10/1 -> din2_10/1, din2_22/1, din2_34/1, din2_46/1
  din1_11/1 -> din2_11/1, din2_23/1, din2_35/1, din2_47/1
  din2_0/1 -> din3_0/1, din3_48/1, din3_96/1
  din2_1/1 -> din3_1/1, din3_49/1, din3_97/1
  din2_2/1 -> din3_2/1, din3_50/1, din3_98/1
  din2_3/1 -> din3_3/1, din3_51/1, din3_99/1
  din2_4/1 -> din3_4/1, din3_52/1, din3_100/1
  din2_5/1 -> din3_5/1, din3_53/1, din3_101/1
  din2_6/1 -> din3_6/1, din3_54/1, din3_102/1
  din2_7/1 -> din3_7/1, din3_55/1, din3_103/1
  din2_8/1 -> din3_8/1, din3_56/1, din3_104/1
  din2_9/1 -> din3_9/1, din3_57/1, din3_105/1
  din2_10/1 -> din3_10/1, din3_58/1, din3_106/1
  din2_11/1 -> din3_11/1, din3_59/1, din3_107/1
  din2_12/1 -> din3_12/1, din3_60/1
  din2_13/1 -> din3_13/1, din3_61/1
  din2_14/1 -> din3_14/1, din3_62/1
  din2_15/1 -> din3_15/1, din3_63/1
  din2_16/1 -> din3_16/1, din3_64/1
  din2_17/1 -> din3_17/1, din3_65/1
  din2_18/1 -> din3_18/1, din3_66/1
  din2_19/1 -> din3_19/1, din3_67/1
  din2_20/1 -> din3_20/1, din3_68/1
  din2_21/1 -> din3_21/1, din3_69/1
  din2_22/1 -> din3_22/1, din3_70/1
  din2_23/1 -> din3_23/1, din3_71/1
  din2_24/1 -> din3_24/1, din3_72/1
  din2_25/1 -> din3_25/1, din3_73/1
  din2_26/1 -> din3_26/1, din3_74/1
  din2_27/1 -> din3_27/1, din3_75/1
  din2_28/1 -> din3_28/1, din3_76/1
  din2_29/1 -> din3_29/1, din3_77/1
  din2_30/1 -> din3_30/1, din3_78/1
  din2_31/1 -> din3_31/1, din3_79/1
  din2_32/1 -> din3_32/1, din3_80/1
  din2_33/1 -> din3_33/1, din3_81/1
  din2_34/1 -> din3_34/1, din3_82/1
  din2_35/1 -> din3_35/1, din3_83/1
  din2_36/1 -> din3_36/1, din3_84/1
  din2_37/1 -> din3_37/1, din3_85/1
  din2_38/1 -> din3_38/1, din3_86/1
  din2_39/1 -> din3_39/1, din3_87/1
  din2_40/1 -> din3_40/1, din3_88/1
  din2_41/1 -> din3_41/1, din3_89/1
  din2_42/1 -> din3_42/1, din3_90/1
  din2_43/1 -> din3_43/1, din3_91/1
  din2_44/1 -> din3_44/1, din3_92/1
  din2_45/1 -> din3_45/1, din3_93/1
  din2_46/1 -> din3_46/1, din3_94/1
  din2_47/1 -> din3_47/1, din3_95/1
  din3_0/1 -> bussify/1(in1)
  din3_1/1 -> bussify/2(in2)
  din3_2/1 -> bussify/3(in3)
  din3_3/1 -> bussify/4(in4)
  din3_4/1 -> bussify/5(in5)
  din3_5/1 -> bussify/6(in6)
  din3_6/1 -> bussify/7(in7)
  din3_7/1 -> bussify/8(in8)
  din3_8/1 -> bussify/9(in9)
  din3_9/1 -> bussify/10(in10)
  din3_10/1 -> bussify/11(in11)
  din3_11/1 -> bussify/12(in12)
  din3_12/1 -> bussify/13(in13)
  din3_13/1 -> bussify/14(in14)
  din3_14/1 -> bussify/15(in15)
  din3_15/1 -> bussify/16(in16)
  din3_16/1 -> bussify/17(in17)
  din3_17/1 -> bussify/18(in18)
  din3_18/1 -> bussify/19(in19)
  din3_19/1 -> bussify/20(in20)
  din3_20/1 -> bussify/21(in21)
  din3_21/1 -> bussify/22(in22)
  din3_22/1 -> bussify/23(in23)
  din3_23/1 -> bussify/24(in24)
  din3_24/1 -> bussify/25(in25)
  din3_25/1 -> bussify/26(in26)
  din3_26/1 -> bussify/27(in27)
  din3_27/1 -> bussify/28(in28)
  din3_28/1 -> bussify/29(in29)
  din3_29/1 -> bussify/30(in30)
  din3_30/1 -> bussify/31(in31)
  din3_31/1 -> bussify/32(in32)
  din3_32/1 -> bussify/33(in33)
  din3_33/1 -> bussify/34(in34)
  din3_34/1 -> bussify/35(in35)
  din3_35/1 -> bussify/36(in36)
  din3_36/1 -> bussify/37(in37)
  din3_37/1 -> bussify/38(in38)
  din3_38/1 -> bussify/39(in39)
  din3_39/1 -> bussify/40(in40)
  din3_40/1 -> bussify/41(in41)
  din3_41/1 -> bussify/42(in42)
  din3_42/1 -> bussify/43(in43)
  din3_43/1 -> bussify/44(in44)
  din3_44/1 -> bussify/45(in45)
  din3_45/1 -> bussify/46(in46)
  din3_46/1 -> bussify/47(in47)
  din3_47/1 -> bussify/48(in48)
  din3_48/1 -> bussify/49(in49)
  din3_49/1 -> bussify/50(in50)
  din3_50/1 -> bussify/51(in51)
  din3_51/1 -> bussify/52(in52)
  din3_52/1 -> bussify/53(in53)
  din3_53/1 -> bussify/54(in54)
  din3_54/1 -> bussify/55(in55)
  din3_55/1 -> bussify/56(in56)
  din3_56/1 -> bussify/57(in57)
  din3_57/1 -> bussify/58(in58)
  din3_58/1 -> bussify/59(in59)
  din3_59/1 -> bussify/60(in60)
  din3_60/1 -> bussify/61(in61)
  din3_61/1 -> bussify/62(in62)
  din3_62/1 -> bussify/63(in63)
  din3_63/1 -> bussify/64(in64)
  din3_64/1 -> bussify/65(in65)
  din3_65/1 -> bussify/66(in66)
  din3_66/1 -> bussify/67(in67)
  din3_67/1 -> bussify/68(in68)
  din3_68/1 -> bussify/69(in69)
  din3_69/1 -> bussify/70(in70)
  din3_70/1 -> bussify/71(in71)
  din3_71/1 -> bussify/72(in72)
  din3_72/1 -> bussify/73(in73)
  din3_73/1 -> bussify/74(in74)
  din3_74/1 -> bussify/75(in75)
  din3_75/1 -> bussify/76(in76)
  din3_76/1 -> bussify/77(in77)
  din3_77/1 -> bussify/78(in78)
  din3_78/1 -> bussify/79(in79)
  din3_79/1 -> bussify/80(in80)
  din3_80/1 -> bussify/81(in81)
  din3_81/1 -> bussify/82(in82)
  din3_82/1 -> bussify/83(in83)
  din3_83/1 -> bussify/84(in84)
  din3_84/1 -> bussify/85(in85)
  din3_85/1 -> bussify/86(in86)
  din3_86/1 -> bussify/87(in87)
  din3_87/1 -> bussify/88(in88)
  din3_88/1 -> bussify/89(in89)
  din3_89/1 -> bussify/90(in90)
  din3_90/1 -> bussify/91(in91)
  din3_91/1 -> bussify/92(in92)
  din3_92/1 -> bussify/93(in93)
  din3_93/1 -> bussify/94(in94)
  din3_94/1 -> bussify/95(in95)
  din3_95/1 -> bussify/96(in96)
  din3_96/1 -> bussify/97(in97)
  din3_97/1 -> bussify/98(in98)
  din3_98/1 -> bussify/99(in99)
  din3_99/1 -> bussify/100(in100)
  din3_100/1 -> bussify/101(in101)
  din3_101/1 -> bussify/102(in102)
  din3_102/1 -> bussify/103(in103)
  din3_103/1 -> bussify/104(in104)
  din3_104/1 -> bussify/105(in105)
  din3_105/1 -> bussify/106(in106)
  din3_106/1 -> bussify/107(in107)
  din3_107/1 -> bussify/108(in108)
  bussify/1(bus_out) -> out/1

== system s_c_nbe_m32k/nb_pfb/pfb_fir_generic1/pfb_fir_taps/tap_delays/rep_wea0 ==
  in : Inport
  bussify : Subsystem  mask(bus_create){inputNum=108}
      mask prompts: inputNum "Number of inputs:"
      mask init:
      | bus_create_init(gcb,...
      |     'inputNum', inputNum);
  out : Outport
  wires:
  in/1 -> bussify/1(in1), bussify/2(in2), bussify/3(in3), bussify/4(in4), bussify/5(in5), bussify/6(in6), bussify/7(in7), bussify/8(in8), bussify/9(in9), bussify/10(in10), bussify/11(in11), bussify/12(in12), bussify/13(in13), bussify/14(in14), bussify/15(in15), bussify/16(in16), bussify/17(in17), bussify/18(in18), bussify/19(in19), bussify/20(in20), bussify/21(in21), bussify/22(in22), bussify/23(in23), bussify/24(in24), bussify/25(in25), bussify/26(in26), bussify/27(in27), bussify/28(in28), bussify/29(in29), bussify/30(in30), bussify/31(in31), bussify/32(in32), bussify/33(in33), bussify/34(in34), bussify/35(in35), bussify/36(in36), bussify/37(in37), bussify/38(in38), bussify/39(in39), bussify/40(in40), bussify/41(in41), bussify/42(in42), bussify/43(in43), bussify/44(in44), bussify/45(in45), bussify/46(in46), bussify/47(in47), bussify/48(in48), bussify/49(in49), bussify/50(in50), bussify/51(in51), bussify/52(in52), bussify/53(in53), bussify/54(in54), bussify/55(in55), bussify/56(in56), bussify/57(in57), bussify/58(in58), bussify/59(in59), bussify/60(in60), bussify/61(in61), bussify/62(in62), bussify/63(in63), bussify/64(in64), bussify/65(in65), bussify/66(in66), bussify/67(in67), bussify/68(in68), bussify/69(in69), bussify/70(in70), bussify/71(in71), bussify/72(in72), bussify/73(in73), bussify/74(in74), bussify/75(in75), bussify/76(in76), bussify/77(in77), bussify/78(in78), bussify/79(in79), bussify/80(in80), bussify/81(in81), bussify/82(in82), bussify/83(in83), bussify/84(in84), bussify/85(in85), bussify/86(in86), bussify/87(in87), bussify/88(in88), bussify/89(in89), bussify/90(in90), bussify/91(in91), bussify/92(in92), bussify/93(in93), bussify/94(in94), bussify/95(in95), bussify/96(in96), bussify/97(in97), bussify/98(in98), bussify/99(in99), bussify/100(in100), bussify/101(in101), bussify/102(in102), bussify/103(in103), bussify/104(in104), bussify/105(in105), bussify/106(in106), bussify/107(in107), bussify/108(in108)
  bussify/1(bus_out) -> out/1
